simulink library "pgctrl"  (R2016b)
settings: Solver=VariableStepAuto  StartTime=0.0  StopTime=10.0  RelTol=1e-3
values from neighbouring files (symbols this model uses):
  pglfd_damping_multiplier = 1.0    (= 1)    [init_pglfd.m]
undefined symbols (not defined in the file or in its folder): curl, DiscIntNeverNeededParam, manifold_stiffness_delay_buffer_size, R3, SO3
libraries: pgctrl x24, pgmanif x15, pgtrafo x10, simulink x8, simulink_need_slupdate x1
(part 1 of 2)
settings Model: Creator=Maximilian  LastModifiedBy=mueh_mm
settings OptimizationCC: LifeSpan=inf
settings DebuggingCC: SFExecutionAtInitializationDiag=none

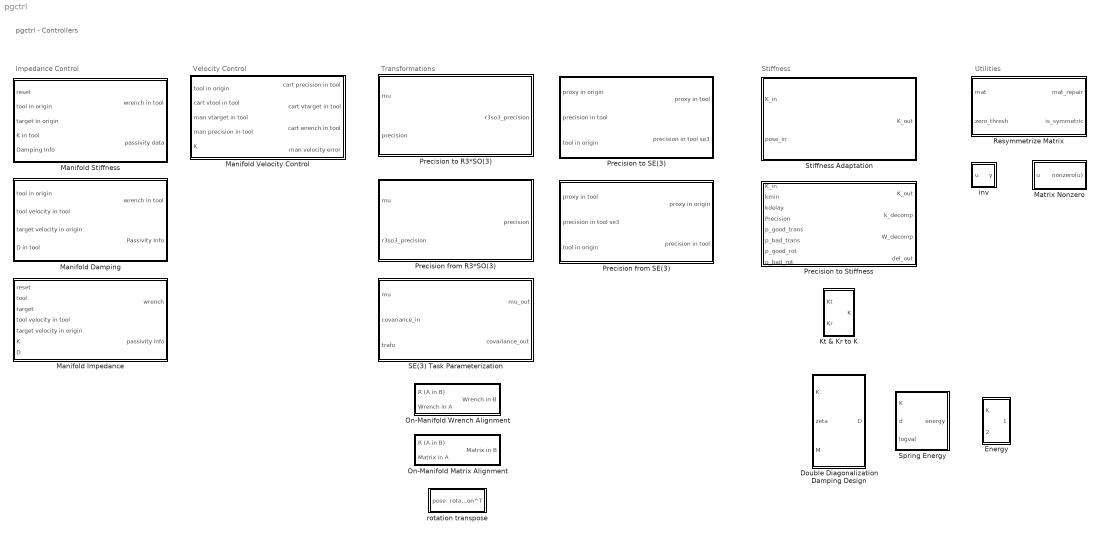
== system pgctrl ==
  note: Impedance Control
  note: pgctrl - Controllers
  note: Transformations
  note: Velocity Control
  note: Utilities
  note: Stiffness
  Double Diagonalization Damping Design : Subsystem
  Energy : Subsystem
  Kt & Kr to K : Subsystem
  Manifold Damping : Subsystem  mask(On-Manifold Damping){manifold_description_damping=R3*SO3, eps_radius=0.02}
      mask prompts: manifold_description_damping "Manifold Description"; eps_radius "Epsilon for Manifold Radius"
      mask help: This block implements the function F = D * v, generalized on the selected manifold.
      mask init:
      | % mask setup
      | mask_styles = get_param(gcb, 'MaskStyles');
      | mask_styles{1} = get_manifold_popup();
      | set_param(gcb, 'MaskStyles', mask_styles);
      | 
      | % set inside manifolds
      | set_param([gcb '/tool To Manifold'], 'manifold_description_raw', manifold_description_damping);
      | set_param([gcb '/Manifold Jacobian'], 'manifold_description_raw', manifold_description_damping);
      mask TypeOptions manifold_description_damping: SO2 | S2 | SO3 | R3*SO3 | SO2*R2*SO3 | S2*R1*SO3
      mask Display:
      | disp(['{\bf\fontsize{12}Damping}' char(10) char(10)], 'texmode','on');
      | disp([char(10) char(10) char(10) char(manifold_description_damping)]);
      | port_label('input', 1, 'tool in origin');
      | port_label('input', 2, 'vtool in tool');
      | port_label('input', 3, 'vtarget in origin');
      | port_label('input', 4, 'D in tool');
      | port_label('output', 1, 'wrench in tool');
      | port_label('output', 2, 'Passivity Info');
  Manifold Impedance : Subsystem  mask(On-Manifold Impedance){manifold_description_impedance=R3*SO3, eps_radius=0.02, passivity_method=None, initial_energy=0, initial_power=0, allow_asymmetric=off, p_active_asym=0, max_increase_passive=10}
      mask prompts: manifold_description_impedance "Manifold Description"; eps_radius "Epsilon for Manifold Radius"; passivity_method "Passivity Method"; initial_energy "Initial Energy (Joule)"; initial_power "Usage rate of initial energy (Watt)"; allow_asymmetric "Allow Asymmetric Part of Stiffness Matrix"; p_active_asym "Active power for asymmetric part"; max_increase_passive "Maximum increase of length per second"
      mask help: This block implements the function F = K * x + D * v, generalized on the selected manifold.
      mask init:
      | % mask setup
      | mask_styles = get_param(gcb, 'MaskStyles');
      | mask_styles{1} = get_manifold_popup();
      | set_param(gcb, 'MaskStyles', mask_styles);
      | 
      | % set inside manifolds
      | set_param([gcb '/Manifold Stiffness'], 'manifold_description_stiffness', manifold_description_impedance);
      | set_param([gcb '/Manifold Damping'], 'manifold_description_damping', manifold_description_impedance);
      | set_param([gcb '/Manifold Curl Stiffness/tool To Manifold'], 'manifold_description_raw', manifold_description_impedance);
      | set_param([gcb '/Manifold Curl Stiffness/Manifold Jacobian'], 'manifold_description_raw', manifold_description_impedance);
      mask TypeOptions manifold_description_impedance: SO2 | S2 | SO3 | R3*SO3 | SO2*R2*SO3 | S2*R1*SO3
      mask TypeOptions passivity_method: None | Limit delta x | Limit Kdot | Limit delta x discrete
      mask Callback passivity_method: set_param([gcb '/Manifold Stiffness'], 'passivity_method', get_param(gcb, 'passivity_method'));
      mask Display:
      | disp(['{\bf\fontsize{12}Impedance}' char(10) char(10)], 'texmode','on');
      | disp([char(10) char(10) char(10) char(manifold_description_impedance)]);
      | port_label('input', 1, 'reset');
      | port_label('input', 2, 'tool in origin');
      | port_label('input', 3, 'target in origin');
      | port_label('input', 4, 'vtool in tool');
      | port_label('input', 5, 'vtarget in origin');
      | port_label('input', 6, 'K in tool');
      | port_label('input', 7, 'D in tool');
      | port_label('output', 1, 'wrench in tool');
      | port_label('output', 2, 'passivity info');
  Manifold Stiffness : Subsystem  mask(On-Manifold Stiffness){manifold_description_stiffness=R3*SO3, eps_radius=0.02, passivity_method=None, initial_energy=0, initial_power=0, max_increase_passive=10}
      mask prompts: manifold_description_stiffness "Manifold Description"; eps_radius "Epsilon for Manifold Radius"; passivity_method "Passivity Method"; initial_energy "Initial Energy (Joule)"; initial_power "Usage rate of initial energy (Watt)"; max_increase_passive "Maximum increase of length per second"
      mask help: This block implements the function F = K * x, generalized on the selected manifold.
      mask init:
      | % mask setup
      | mask_styles = get_param(gcb, 'MaskStyles');
      | mask_styles{1} = get_manifold_popup();
      | set_param(gcb, 'MaskStyles', mask_styles);
      | 
      | % set inside manifolds
      | set_param([gcb '/target To Manifold'], 'manifold_description_raw', manifold_description_stiffness);
      | set_param([gcb '/tool To Manifold'], 'manifold_description_raw', manifold_description_stiffness);
      | set_param([gcb '/Manifold Jacobian'], 'manifold_description_raw', manifold_description_stiffness);
      | set_param([gcb '/Manifold Log'], 'manifold_description_raw', manifold_description_stiffness);
      mask TypeOptions manifold_description_stiffness: SO2 | S2 | SO3 | R3*SO3 | SO2*R2*SO3 | S2*R1*SO3
      mask TypeOptions passivity_method: None | Limit delta x | Limit Kdot | Limit delta x discrete
      mask Display:
      | disp(['{\bf\fontsize{12}Stiffness}' char(10) char(10)], 'texmode','on');
      | disp([char(10) char(10) char(10) char(manifold_description_stiffness)]);
      | port_label('input', 1, 'reset');
      | port_label('input', 2, 'tool in origin');
      | port_label('input', 3, 'target in origin');
      | port_label('input', 4, 'K in tool');
      | port_label('input', 5, 'Damping Info');
      | port_label('output', 1, 'wrench in tool');
      | port_label('output', 2, 'passivity info');
  Manifold Velocity Control : Subsystem  mask(On-Manifold Velocity Control){manifold_description_stiffness=R3*SO3, eps_radius=0.02}
      mask prompts: manifold_description_stiffness "Manifold Description"; eps_radius "Epsilon for Manifold Radius"
      mask help: This block implements the function F = K * (xref' - x'), generalized on the selected manifold. It outputs a cartesian wrench in the target frame
      mask init:
      | % mask setup
      | mask_styles = get_param(gcb, 'MaskStyles');
      | mask_styles{1} = get_manifold_popup();
      | set_param(gcb, 'MaskStyles', mask_styles);
      | 
      | % set inside manifolds
      | set_param([gcb '/tool To Manifold'], 'manifold_description_raw', manifold_description_stiffness);
      | set_param([gcb '/Manifold Jacobian'], 'manifold_description_raw', manifold_description_stiffness);
      | set_param([gcb '/Precision to SE(3)'], 'manifold_description_raw', manifold_description_stiffness);
      | set_param([gcb '/Stiffness Adaptation'], 'manifold_description_raw', manifold_description_stiffness);
      mask TypeOptions manifold_description_stiffness: SO2 | S2 | SO3 | R3*SO3 | SO2*R2*SO3 | S2*R1*SO3
      mask Display:
      | disp(['{\bf\fontsize{12}Velocity Control}' char(10) char(10)], 'texmode','on');
      | disp([char(10) char(10) char(10) char(manifold_description_stiffness)]);
      | port_label('input', 1, 'tool in origin');
      | port_label('input', 2, 'cart vtool');
      | port_label('input', 3, 'man vtarget');
      | port_label('input', 4, 'man prec');
      | port_label('input', 5, 'D');
      | port_label('output', 1, 'cart precision');
      | port_label('output', 2, 'cart vtarget');
      | port_label('output', 3, 'cart wrench');
      | port_label('output', 4, 'man velocity error');
  Matrix Nonzero : Subsystem
  On-Manifold Matrix Alignment : Subsystem
  On-Manifold Wrench Alignment : Subsystem
  Precision from R3*SO(3) : Subsystem  mask(Precision from R3*SO(3)){manifold_description_raw=R3*SO3, eps_radius=0.02}
      mask prompts: manifold_description_raw "Manifold Description"; eps_radius "Epsilon for Manifold Radius"
      mask help: This block transforms a covariance matrix from R3*SO3 to a covariance matrix on the selected manifold using the jacobian.
      mask init:
      | % mask setup
      | mask_styles = get_param(gcb, 'MaskStyles');
      | mask_styles{1} = get_manifold_popup();
      | set_param(gcb, 'MaskStyles', mask_styles);
      | 
      | % set inside manifolds
      | set_param([gcb '/To Manifold'], 'manifold_description_raw', manifold_description_raw);
      | set_param([gcb '/Manifold Jacobian'], 'manifold_description_raw', manifold_description_raw);
      mask TypeOptions manifold_description_raw: SO2 | S2 | SO3 | R3*SO3 | SO2*R2*SO3 | S2*R1*SO3
      mask Display:
      | text(0.5, 0.7, ['{\bf\fontsize{12}' char(manifold_description_raw) char(10) 'Precision}'], 'HorizontalAlignment', 'center', 'texmode', 'on');
      | disp([char(10) char(10) char(10) 'from R3*SO3']);
      | port_label('input', 1, 'mu');
      | port_label('input', 2, 'R3*SO(3) precision');
      | port_label('output', 1, 'precision');
  Precision from SE(3) : Subsystem  mask(Precision from SE(3)){manifold_description_raw=R3*SO3, eps_radius=0.02}
      mask prompts: manifold_description_raw "Manifold Description"; eps_radius "Epsilon for Manifold Radius"
      mask help: Transform a SE(3) precision matrix in tool coordinates at proxy to an on-manifold precision matrix in origin coordinates.
      mask init:
      | % mask setup
      | mask_styles = get_param(gcb, 'MaskStyles');
      | mask_styles{1} = get_manifold_popup();
      | set_param(gcb, 'MaskStyles', mask_styles);
      | 
      | % set inside manifolds
      | set_param([gcb '/Precision from R3*SO(3)'], 'manifold_description_raw', manifold_description_raw);
      mask TypeOptions manifold_description_raw: SO2 | S2 | SO3 | R3*SO3 | SO2*R2*SO3 | S2*R1*SO3
      mask Display:
      | text(0.5, 0.7, ['{\bf\fontsize{12}' char(manifold_description_raw) char(10) 'Precision}'], 'HorizontalAlignment', 'center', 'texmode', 'on');
      | disp([char(10) char(10) char(10) 'from SE(3)']);
      | port_label('input', 1, 'proxy in tool');
      | port_label('input', 2, 'precision in tool se(3)');
      | port_label('input', 3, 'tool in origin');
      | port_label('output', 1, 'proxy in origin');
      | port_label('output', 2, 'precision in tool');
  Precision to R3*SO(3) : Subsystem  mask(Precision to R3*SO(3)){manifold_description_raw=R3*SO3, eps_radius=0.02}
      mask prompts: manifold_description_raw "Manifold Description"; eps_radius "Epsilon for Manifold Radius"
      mask help: This block transforms a covariance matrix on the selected manifold to a R3*SO3 covariance matrix using the jacobian.
      mask init: same as pgctrl/Precision from R3*SO(3)
      mask TypeOptions manifold_description_raw: SO2 | S2 | SO3 | R3*SO3 | SO2*R2*SO3 | S2*R1*SO3
      mask Display:
      | text(0.5, 0.7, ['{\bf\fontsize{12}R3*SO(3)' char(10) 'Precision}'], 'HorizontalAlignment', 'center', 'texmode', 'on');
      | disp([char(10) char(10) char(10) 'from ' char(manifold_description_raw)]);
      | port_label('input', 1, 'mu');
      | port_label('input', 2, 'precision');
      | port_label('output', 1, 'R3*SO(3) precision');
  Precision to SE(3) : Subsystem  mask(Precision to SE(3)){manifold_description_raw=R3*SO3, eps_radius=0.02}
      mask prompts: manifold_description_raw "Manifold Description"; eps_radius "Epsilon for Manifold Radius"
      mask help: Transform an on-manifold precision matrix in origin coordinates at proxy to a SE(3) precision matrix in tool coordinates.
      mask init:
      | % mask setup
      | mask_styles = get_param(gcb, 'MaskStyles');
      | mask_styles{1} = get_manifold_popup();
      | set_param(gcb, 'MaskStyles', mask_styles);
      | 
      | % set inside manifolds
      | set_param([gcb '/Precision to R3*SO(3)'], 'manifold_description_raw', manifold_description_raw);
      mask TypeOptions manifold_description_raw: SO2 | S2 | SO3 | R3*SO3 | SO2*R2*SO3 | S2*R1*SO3
      mask Display:
      | text(0.5, 0.7, ['{\bf\fontsize{12}SE(3)' char(10) 'Precision}'], 'HorizontalAlignment', 'center', 'texmode', 'on');
      | disp([char(10) char(10) char(10) 'from ' char(manifold_description_raw)]);
      | port_label('input', 1, 'proxy in origin');
      | port_label('input', 2, 'precision in tool');
      | port_label('input', 3, 'tool in origin');
      | port_label('output', 1, 'proxy in tool');
      | port_label('output', 2, 'precision in tool se(3)');
  Precision to Stiffness : Subsystem  mask(Precision to Stiffness){}
      mask help: This block decomposes a precision matrix to create a stiffness matrix respecting limits.
      mask Display:
      | disp(['{\bf\fontsize{12}Precision to Stiffness}' char(10) char(10)], 'texmode','on');
      | port_label('input', 1, 'K_{diag}', 'texmode', 'on');
      | port_label('input', 2, 'k_{min}', 'texmode', 'on');
      | port_label('input', 3, 'k_{delay}', 'texmode', 'on');
      | port_label('input', 4, 'Precision');
      | port_label('input', 5, 'P_{good, trans}', 'texmode', 'on');
      | port_label('input', 6, 'P_{bad, trans}', 'texmode', 'on');
      | port_label('input', 7, 'P_{good, rot}', 'texmode', 'on');
      | port_label('input', 8, 'P_{bad, rot}', 'texmode', 'on');
      | port_label('output', 1, 'K_{adapted}', 'texmode', 'on');
      | port_label('output', 2, 'k_{decomp}', 'texmode', 'on');
      | port_label('output', 3, 'W_{decomp}', 'texmode', 'on');
      | port_label('output', 4, 'is_delay');
  Resymmetrize Matrix : MATLAB Function  TreatAsAtomicUnit=on
  SE(3) Task Parameterization : Subsystem  mask(SE(3) Task Parameterization){}
      mask help: This block transports a mean and covariance on R3*SO3 extracted in one coordinate system to another one using the SE(3) transformation trafo.
      mask Display:
      | disp(['{\bf\fontsize{12}SE(3) Task}' char(10) char(10)], 'texmode','on');
      | disp([char(10) char(10) '{\bf\fontsize{12}Parameterization}'], 'texmode','on');
      | port_label('input', 1, 'mu');
      | port_label('input', 2, 'covariance');
      | port_label('input', 3, 'trafo');
      | port_label('output', 1, 'mu');
      | port_label('output', 2, 'covariance');
  Spring Energy : Subsystem
  Stiffness Adaptation : Subsystem  mask(On-Manifold Stiffness Adaptation){manifold_description_raw=R3*SO3, manifold_description=0, manifold_id=0}
      mask prompts: manifold_description_raw "Manifold Description"
      mask help:
      | This block adapts a stiffness matrix on cylindrical or spherical manifolds to ensure stiffness doesn't get too low / too high for the rotational DoF's. Stiffness equivalent to the euclidean case with r=1 is achieved.
      |
      | Note that only diagonal stiffness matrices are supported.
      mask init:
      | % mask setup
      | mask_styles = get_param(gcb, 'MaskStyles');
      | mask_styles{1} = get_manifold_popup();
      | set_param(gcb, 'MaskStyles', mask_styles);
      | 
      | % set description
      | manifold_description = uint8(manifold_description_raw);
      | 
      | % set manifold id
      | manifold_id = 0;
      | if contains(char(manifold_description), 'SO2*R2')
      |     manifold_id = 1;
      | elseif contains(char(manifold_description), 'S2*R1')
      |     manifold_id = 2;
      | end
      mask TypeOptions manifold_description_raw: SO2 | S2 | SO3 | R3*SO3 | SO2*R2*SO3 | S2*R1*SO3
      mask Display:
      | disp(['{\bf\fontsize{12}Stiffness Adaptation}' char(10) char(10)], 'texmode','on');
      | disp([char(10) char(10) char(10) char(manifold_description)]);
      | port_label('input', 1, 'K');
      | port_label('input', 2, 'pose on manifold');
      | port_label('output', 1, 'K_{adapted}', 'texmode', 'on');
  inv : MATLAB Function  TreatAsAtomicUnit=on
  rotation transpose : Subsystem

== system pgctrl/Double Diagonalization Damping Design ==
  note: ToDo: check if M is PD
  K : Inport
  zeta : Inport  Port=2
  M : Inport  Port=3
  Constant : Constant  Value=zeros(6,6)
  Damping Design using Double Diagonalization : Subsystem
  Logical Operator : Logic  AllPortsSameDT=off  OutDataTypeStr=boolean
  Switch : Switch  Criteria=u2 > Threshold
  check finite : Subsystem
  check symmetric : Subsystem
  symmetrize : Subsystem
  D : Outport
  wires:
  check finite/1(finite) -> Logical Operator/1
  Switch/1 -> D/1
  Constant/1 -> Switch/3
  Logical Operator/1 -> Switch/2
  Damping Design using Double Diagonalization/1(D) -> Switch/1, check finite/1(matrix)
  K/1 -> symmetrize/1(K)
  check symmetric/1(is sym) -> Logical Operator/2
  M/1 -> Damping Design using Double Diagonalization/3(M), check symmetric/1(M)
  zeta/1 -> Damping Design using Double Diagonalization/2(zeta)
  symmetrize/1(Ksym) -> Damping Design using Double Diagonalization/1(K)

== system pgctrl/Energy ==
  K : Inport
  logval : Inport  Port=2
  Constant2 : Constant  Value=0.5
  Math Function2 : Math  Operator=transpose  SaturateOnIntegerOverflow=on
  Product3 : Product  Inputs=4  Multiplication=Matrix(*)
  energy : Outport
  wires:
  Math Function2/1 -> Product3/2
  Product3/1 -> energy/1
  logval/1 -> Math Function2/1, Product3/4
  K/1 -> Product3/3
  Constant2/1 -> Product3/1

== system pgctrl/Kt & Kr to K ==
  Kt : Inport
  Kr : Inport  Port=2
  Empty Stiffness : Constant  Value=zeros(6,6)
  Kr Assignment : Assignment  NumberOfDimensions=2  DiagnosticForDimensions=Warning  IndexOptions=Index vector (dialog),Index vector (dialog)  Indices=4:6,4:6  OutputSizes=1,1
  Kt Assignment : Assignment  NumberOfDimensions=2  DiagnosticForDimensions=Warning  IndexOptions=Index vector (dialog),Index vector (dialog)  Indices=1:3,1:3  OutputSizes=1,1
  K : Outport
  wires:
  Kt Assignment/1 -> Kr Assignment/1
  Kr/1 -> Kr Assignment/2
  Kr Assignment/1 -> K/1
  Kt/1 -> Kt Assignment/2
  Empty Stiffness/1 -> Kt Assignment/1

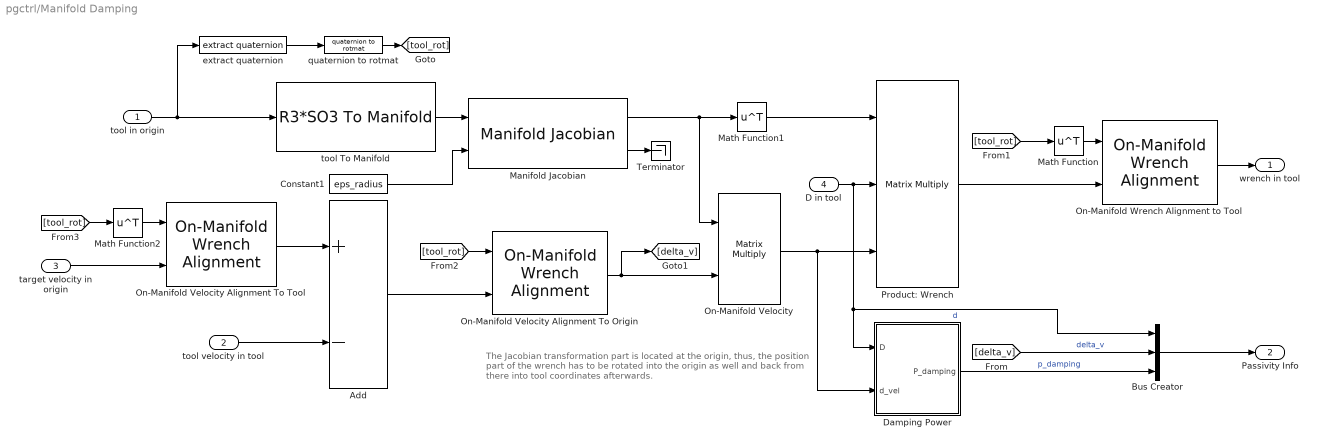
== system pgctrl/Manifold Damping ==
  note: The Jacobian transformation part is located at the origin, thus,
      | the position part of the wrench has to be rotated into the origin as well
      | and back from there into tool coordinates afterwards.
  tool in origin : Inport
  tool velocity in tool : Inport  Port=2
  target velocity in origin : Inport  Port=3
  D in tool : Inport  Port=4
  Add : Sum  Inputs=+-
  Bus Creator : BusCreator  Inputs=3
  Constant1 : Constant  Value=eps_radius
  Damping Power : Subsystem
  Manifold Jacobian : pgmanif/Manifold Jacobian  manifold_description_raw=R3*SO3  manifold_description=0  dim_manifold=0  dim_tangent=0  manifold_id=0
  Math Function : Math  Operator=transpose  SaturateOnIntegerOverflow=on
  Math Function1 : Math  Operator=transpose  SaturateOnIntegerOverflow=on
  Math Function2 : Math  Operator=transpose  SaturateOnIntegerOverflow=on
  On-Manifold Velocity : Product  Multiplication=Matrix(*)
  On-Manifold Velocity Alignment To Origin : pgctrl/On-Manifold Wrench Alignment
  On-Manifold Velocity Alignment To Tool : pgctrl/On-Manifold Wrench Alignment
  On-Manifold Wrench Alignment to Tool : pgctrl/On-Manifold Wrench Alignment
  Product: Wrench : Product  Inputs=3  Multiplication=Matrix(*)
  Terminator : Terminator
  extract quaternion : pgtrafo/extract quaternion
  quaternion to rotmat : pgtrafo/quaternion to rotmat
  tool To Manifold : pgmanif/R3*SO3 To Manifold  manifold_description_raw=R3*SO3  manifold_description=0  dim_manifold=0  dim_tangent=0
  wrench in tool : Outport
  Passivity Info : Outport  Port=2  OutDataTypeStr=Bus: bus_manifold_passivity_damping
  wires:
  tool To Manifold/1 -> Manifold Jacobian/1
  On-Manifold Wrench Alignment to Tool/1 -> wrench in tool/1
  D in tool/1 -> Bus Creator/1, Damping Power/1(D), Product: Wrench/2  "d"
  Manifold Jacobian/1 -> On-Manifold Velocity/1, Math Function1/1
  tool in origin/1 -> extract quaternion/1, tool To Manifold/1
  On-Manifold Velocity Alignment To Tool/1 -> Add/1
  [tool_rot] -> Math Function2/1
  tool velocity in tool/1 -> Add/2
  target velocity in origin/1 -> On-Manifold Velocity Alignment To Tool/2
  Product: Wrench/1 -> On-Manifold Wrench Alignment to Tool/2
  Math Function/1 -> On-Manifold Wrench Alignment to Tool/1
  [tool_rot] -> Math Function/1
  On-Manifold Velocity Alignment To Origin/1 -> [delta_v], On-Manifold Velocity/2
  [tool_rot] -> On-Manifold Velocity Alignment To Origin/1
  Add/1 -> On-Manifold Velocity Alignment To Origin/2
  quaternion to rotmat/1 -> [tool_rot]
  extract quaternion/1 -> quaternion to rotmat/1
  On-Manifold Velocity/1 -> Damping Power/2(d_vel), Product: Wrench/3
  Math Function1/1 -> Product: Wrench/1
  Constant1/1 -> Manifold Jacobian/2
  Manifold Jacobian/2 -> Terminator/1
  Damping Power/1(P_damping) -> Bus Creator/3  "p_damping"
  Bus Creator/1 -> Passivity Info/1
  [delta_v] -> Bus Creator/2  "delta_v"
  Math Function2/1 -> On-Manifold Velocity Alignment To Tool/1

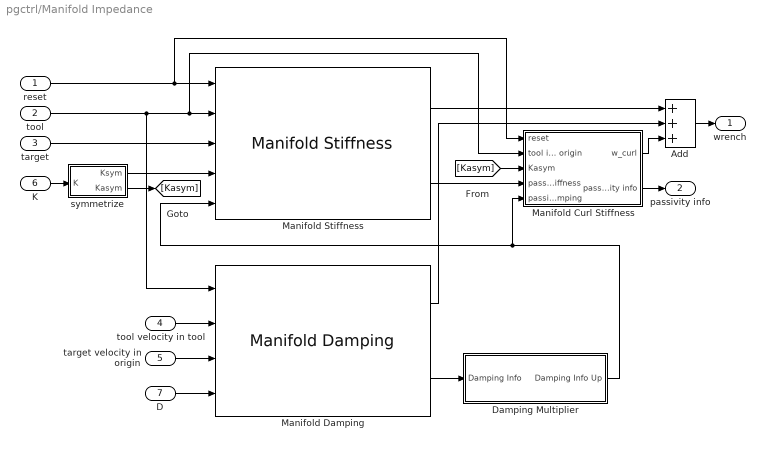
== system pgctrl/Manifold Impedance ==
  reset : Inport
  tool : Inport  Port=2
  target : Inport  Port=3
  tool velocity in tool : Inport  Port=4
  target velocity in origin : Inport  Port=5
  K : Inport  Port=6
  D : Inport  Port=7
  Add : Sum  Inputs=+++
  Damping Multiplier : Subsystem
  Manifold Curl Stiffness : Subsystem
  Manifold Damping : pgctrl/Manifold Damping  manifold_description_damping=R3*SO3  eps_radius=eps_radius
  Manifold Stiffness : pgctrl/Manifold Stiffness  manifold_description_stiffness=R3*SO3  eps_radius=eps_radius  passivity_method=None  initial_energy=initial_energy  initial_power=initial_power  max_increase_passive=max_increase_passive
  symmetrize : Subsystem
  wrench : Outport
  passivity info : Outport  Port=2
  wires:
  Manifold Stiffness/1 -> Add/1
  Manifold Damping/1 -> Add/2
  Add/1 -> wrench/1
  tool/1 -> Manifold Curl Stiffness/2(tool in origin), Manifold Stiffness/2, Manifold Damping/1
  tool velocity in tool/1 -> Manifold Damping/2
  target velocity in origin/1 -> Manifold Damping/3
  D/1 -> Manifold Damping/4
  K/1 -> symmetrize/1(K)
  target/1 -> Manifold Stiffness/3
  reset/1 -> Manifold Curl Stiffness/1(reset), Manifold Stiffness/1
  Manifold Stiffness/2 -> Manifold Curl Stiffness/4(passivity_stiffness)
  Manifold Damping/2 -> Damping Multiplier/1(Damping Info)
  Damping Multiplier/1(Damping Info Up) -> Manifold Stiffness/5, Manifold Curl Stiffness/5(passivity_damping)
  symmetrize/1(Ksym) -> Manifold Stiffness/4
  symmetrize/2(Kasym) -> [Kasym]
  Manifold Curl Stiffness/1(w_curl) -> Add/3
  [Kasym] -> Manifold Curl Stiffness/3(Kasym)
  Manifold Curl Stiffness/2(passivity info) -> passivity info/1

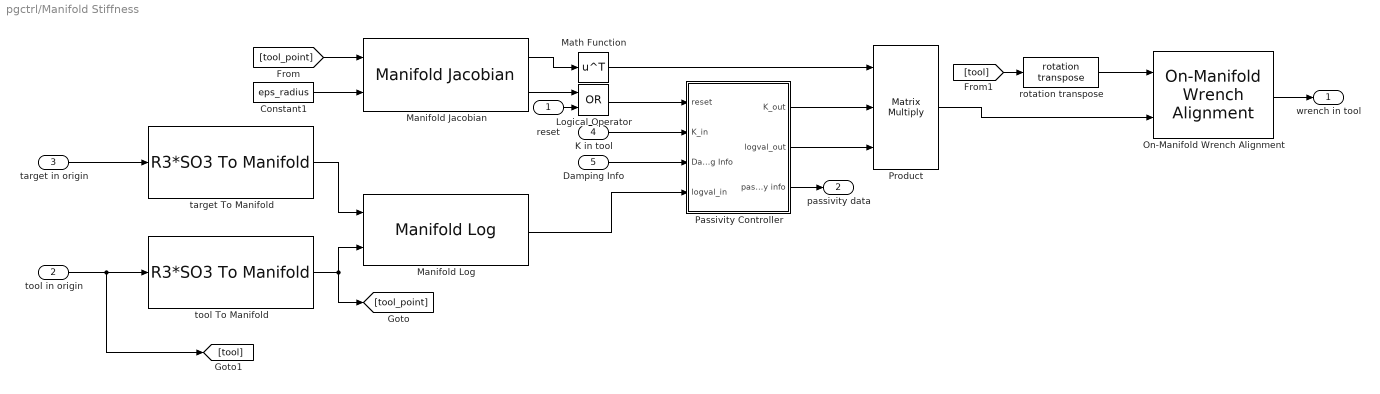
== system pgctrl/Manifold Stiffness ==
  reset : Inport
  tool in origin : Inport  Port=2
  target in origin : Inport  Port=3
  K in tool : Inport  Port=4
  Damping Info : Inport  Port=5  OutDataTypeStr=Bus: bus_manifold_passivity_damping
  Constant1 : Constant  Value=eps_radius
  Logical Operator : Logic  Operator=OR  AllPortsSameDT=off  OutDataTypeStr=boolean
  Manifold Jacobian : pgmanif/Manifold Jacobian  manifold_description_raw=R3*SO3  manifold_description=0  dim_manifold=0  dim_tangent=0  manifold_id=0
  Manifold Log : pgmanif/Manifold Log  manifold_description_raw=R3*SO3  manifold_description=0  dim_manifold=0  dim_tangent=0
  Math Function : Math  Operator=transpose  SaturateOnIntegerOverflow=on
  On-Manifold Wrench Alignment : pgctrl/On-Manifold Wrench Alignment
  Passivity Controller : Subsystem
  Product : Product  Inputs=3  Multiplication=Matrix(*)
  rotation transpose : pgctrl/rotation transpose
  target To Manifold : pgmanif/R3*SO3 To Manifold  manifold_description_raw=R3*SO3  manifold_description=0  dim_manifold=0  dim_tangent=0
  tool To Manifold : pgmanif/R3*SO3 To Manifold  manifold_description_raw=R3*SO3  manifold_description=0  dim_manifold=0  dim_tangent=0
  wrench in tool : Outport
  passivity data : Outport  Port=2
  wires:
  Product/1 -> On-Manifold Wrench Alignment/2
  target To Manifold/1 -> Manifold Log/1
  tool To Manifold/1 -> [tool_point], Manifold Log/2
  [tool_point] -> Manifold Jacobian/1
  Manifold Jacobian/1 -> Math Function/1
  target in origin/1 -> target To Manifold/1
  tool in origin/1 -> tool To Manifold/1, [tool]
  On-Manifold Wrench Alignment/1 -> wrench in tool/1
  [tool] -> rotation transpose/1
  rotation transpose/1 -> On-Manifold Wrench Alignment/1
  Math Function/1 -> Product/1
  Constant1/1 -> Manifold Jacobian/2
  K in tool/1 -> Passivity Controller/2(K_in)
  Damping Info/1 -> Passivity Controller/3(Damping Info)
  Manifold Log/1 -> Passivity Controller/4(logval_in)
  Passivity Controller/1(K_out) -> Product/2
  Passivity Controller/2(logval_out) -> Product/3
  Manifold Jacobian/2 -> Logical Operator/1
  Logical Operator/1 -> Passivity Controller/1(reset)
  reset/1 -> Logical Operator/2
  Passivity Controller/3(passivity info) -> passivity data/1

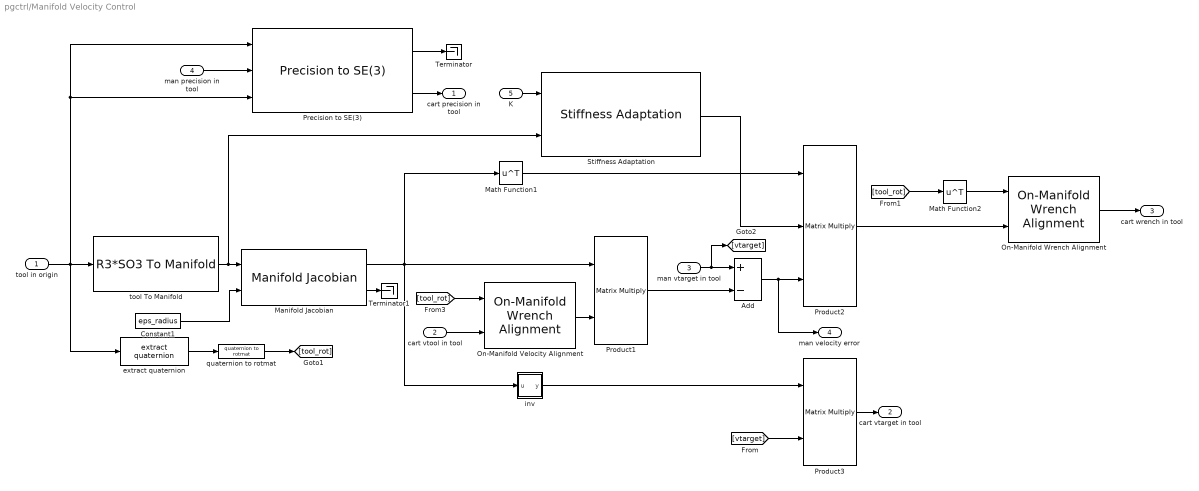
== system pgctrl/Manifold Velocity Control ==
  tool in origin : Inport
  cart vtool in tool : Inport  Port=2
  man vtarget in tool : Inport  Port=3
  man precision in tool : Inport  Port=4
  K : Inport  Port=5
  Add : Sum  Inputs=+-
  Constant1 : Constant  Value=eps_radius
  Manifold Jacobian : pgmanif/Manifold Jacobian  manifold_description_raw=R3*SO3  manifold_description=0  dim_manifold=0  dim_tangent=0  manifold_id=0
  Math Function1 : Math  Operator=transpose  SaturateOnIntegerOverflow=on
  Math Function2 : Math  Operator=transpose  SaturateOnIntegerOverflow=on
  On-Manifold Velocity Alignment : pgctrl/On-Manifold Wrench Alignment
  On-Manifold Wrench Alignment : pgctrl/On-Manifold Wrench Alignment
  Precision to SE(3) : pgctrl/Precision to SE(3)  manifold_description_raw=R3*SO3  eps_radius=eps_radius
  Product1 : Product  Multiplication=Matrix(*)
  Product2 : Product  Inputs=3  Multiplication=Matrix(*)
  Product3 : Product  Multiplication=Matrix(*)
  Stiffness Adaptation : pgctrl/Stiffness Adaptation  manifold_description_raw=R3*SO3  manifold_description=0  manifold_id=0
  Terminator : Terminator
  Terminator1 : Terminator
  extract quaternion : pgtrafo/extract quaternion
  inv : MATLAB Function  TreatAsAtomicUnit=on
  quaternion to rotmat : pgtrafo/quaternion to rotmat
  tool To Manifold : pgmanif/R3*SO3 To Manifold  manifold_description_raw=R3*SO3  manifold_description=0  dim_manifold=0  dim_tangent=0
  cart precision in tool : Outport
  cart vtarget in tool : Outport  Port=2
  cart wrench in tool : Outport  Port=3
  man velocity error : Outport  Port=4
  wires:
  [tool_rot] -> Math Function2/1
  On-Manifold Wrench Alignment/1 -> cart wrench in tool/1
  tool To Manifold/1 -> Manifold Jacobian/1, Stiffness Adaptation/2
  Manifold Jacobian/1 -> inv/1(u), Math Function1/1, Product1/1
  Product1/1 -> Add/2
  man vtarget in tool/1 -> [vtarget], Add/1
  Add/1 -> man velocity error/1, Product2/3
  Product2/1 -> On-Manifold Wrench Alignment/2
  [vtarget] -> Product3/2
  Product3/1 -> cart vtarget in tool/1
  man precision in tool/1 -> Precision to SE(3)/2
  Precision to SE(3)/2 -> cart precision in tool/1
  tool in origin/1 -> tool To Manifold/1, extract quaternion/1, Precision to SE(3)/3, Precision to SE(3)/1
  [tool_rot] -> On-Manifold Velocity Alignment/1
  cart vtool in tool/1 -> On-Manifold Velocity Alignment/2
  On-Manifold Velocity Alignment/1 -> Product1/2
  extract quaternion/1 -> quaternion to rotmat/1
  quaternion to rotmat/1 -> [tool_rot]
  K/1 -> Stiffness Adaptation/1
  Stiffness Adaptation/1 -> Product2/2
  Precision to SE(3)/1 -> Terminator/1
  Math Function1/1 -> Product2/1
  inv/1(y) -> Product3/1
  Constant1/1 -> Manifold Jacobian/2
  Math Function2/1 -> On-Manifold Wrench Alignment/1
  Manifold Jacobian/2 -> Terminator1/1

== system pgctrl/Matrix Nonzero ==
  note: Check if any of the Matrix entries is nonzero.
  u : Inport
  Matrix Nonzero : MATLAB Function  TreatAsAtomicUnit=on
  nonzero(u) : Outport
  wires:
  Matrix Nonzero/1(y) -> nonzero(u)/1
  u/1 -> Matrix Nonzero/1(u)

== system pgctrl/On-Manifold Matrix Alignment ==
  note: When computing an on-manifold matrix in a different coordinate system,
      | the positional part must be rotated accordingly: M_in_B = [R,0;0,I] M_in_A [R',0;0,I]
  R (A in B) : Inport
  Matrix in A : Inport  Port=2
  Assignment : Assignment  NumberOfDimensions=2  DiagnosticForDimensions=Warning  IndexOptions=Index vector (dialog),Index vector (dialog)  Indices=1:3,1:3  OutputSizes=1,1
  Constant : Constant  Value=eye(6)
  Math Function : Math  Operator=transpose  SaturateOnIntegerOverflow=on
  Product : Product  Inputs=3  Multiplication=Matrix(*)
  Matrix in B : Outport
  wires:
  Assignment/1 -> Math Function/1, Product/1
  R (A in B)/1 -> Assignment/2
  Constant/1 -> Assignment/1
  Product/1 -> Matrix in B/1
  Matrix in A/1 -> Product/2
  Math Function/1 -> Product/3

== system pgctrl/On-Manifold Wrench Alignment ==
  note: When computing an on-manifold wrench in a different coordinate system,
      | the forces must be rotated accordingly.
  R (A in B) : Inport
  Wrench in A : Inport  Port=2
  Product : Product  Multiplication=Matrix(*)
  Selector : Selector  InputPortWidth=6  IndexOptions=Index vector (dialog)  Indices=1:3  OutputSizes=1
  Selector1 : Selector  InputPortWidth=6  IndexOptions=Index vector (dialog)  Indices=4:6  OutputSizes=1
  Vector Concatenate : Concatenate
  Wrench in B : Outport
  wires:
  Wrench in A/1 -> Selector1/1, Selector/1
  Vector Concatenate/1 -> Wrench in B/1
  Selector/1 -> Product/2
  Selector1/1 -> Vector Concatenate/2
  Product/1 -> Vector Concatenate/1
  R (A in B)/1 -> Product/1

== system pgctrl/Precision from R3*SO(3) ==
  mu : Inport
  r3so3_precision : Inport  Port=2
  Constant1 : Constant  Value=eps_radius
  Manifold Jacobian : pgmanif/Manifold Jacobian  manifold_description_raw=R3*SO3  manifold_description=0  dim_manifold=0  dim_tangent=0  manifold_id=0
  Math Function : Math  Operator=transpose  SaturateOnIntegerOverflow=on
  Product : Product  Inputs=3  Multiplication=Matrix(*)
  To Manifold : pgmanif/R3*SO3 To Manifold  manifold_description_raw=R3*SO3  manifold_description=0  dim_manifold=0  dim_tangent=0
  inverse : MATLAB Function  TreatAsAtomicUnit=on
  precision : Outport
  wires:
  r3so3_precision/1 -> Product/2
  To Manifold/1 -> Manifold Jacobian/1
  mu/1 -> To Manifold/1
  Product/1 -> precision/1
  inverse/1(y) -> Product/1
  Manifold Jacobian/1 -> Math Function/1
  Math Function/1 -> inverse/2(u), Product/3
  Constant1/1 -> Manifold Jacobian/2
  Manifold Jacobian/2 -> inverse/1(singular)

== system pgctrl/Precision from SE(3) ==
  note: SE(3) task parametrization is needed to transform from tool to origin.
  note: Convert the precision matrix to manifold tangent coordinates from R3*SO3
      | using the manifold Jacobian.
  note: Some later calculations depend on whether the covariance is truly zero.
  proxy in tool : Inport
  precision in tool se3 : Inport  Port=2
  tool in origin : Inport  Port=3
  Constant : Constant  Value=zeros(6,6)
  Matrix Nonzero : pgctrl/Matrix Nonzero
  Precision from R3*SO(3) : pgctrl/Precision from R3*SO(3)  manifold_description_raw=R3*SO3  eps_radius=eps_radius
  SE(3) Task Parameterization : pgctrl/SE(3) Task Parameterization
  Switch : Switch  Criteria=u2 > Threshold
  proxy in origin : Outport
  precision in tool : Outport  Port=2
  wires:
  SE(3) Task Parameterization/1 -> Precision from R3*SO(3)/1, proxy in origin/1
  proxy in tool/1 -> SE(3) Task Parameterization/1
  tool in origin/1 -> SE(3) Task Parameterization/3
  Constant/1 -> Switch/3
  precision in tool se3/1 -> Matrix Nonzero/1, SE(3) Task Parameterization/2
  Matrix Nonzero/1 -> Switch/2
  Switch/1 -> precision in tool/1
  SE(3) Task Parameterization/2 -> Precision from R3*SO(3)/2
  Precision from R3*SO(3)/1 -> Switch/1

== system pgctrl/Precision to R3*SO(3) ==
  mu : Inport
  precision : Inport  Port=2
  Constant1 : Constant  Value=eps_radius
  Manifold Jacobian : pgmanif/Manifold Jacobian  manifold_description_raw=R3*SO3  manifold_description=0  dim_manifold=0  dim_tangent=0  manifold_id=0
  Math Function : Math  Operator=transpose  SaturateOnIntegerOverflow=on
  Product : Product  Inputs=3  Multiplication=Matrix(*)
  Terminator : Terminator
  To Manifold : pgmanif/R3*SO3 To Manifold  manifold_description_raw=R3*SO3  manifold_description=0  dim_manifold=0  dim_tangent=0
  r3so3_precision : Outport
  wires:
  Product/1 -> r3so3_precision/1
  mu/1 -> To Manifold/1
  To Manifold/1 -> Manifold Jacobian/1
  precision/1 -> Product/2
  Manifold Jacobian/1 -> Product/3, Math Function/1
  Math Function/1 -> Product/1
  Constant1/1 -> Manifold Jacobian/2
  Manifold Jacobian/2 -> Terminator/1

== system pgctrl/Precision to SE(3) ==
  note: Some later calculations depend on whether the covariance is truly zero.
  note: Convert the precision matrix from manifold tangent coordinates to R3*SO3
      | using the manifold Jacobian.
  note: SE(3) task parametrization is needed as the fixture arbitration happens in the toolframe.
  proxy in origin : Inport
  precision in tool : Inport  Port=2
  tool in origin : Inport  Port=3
  Constant : Constant  Value=zeros(6,6)
  Matrix Nonzero : pgctrl/Matrix Nonzero
  Precision to R3*SO(3) : pgctrl/Precision to R3*SO(3)  manifold_description_raw=R3*SO3  eps_radius=eps_radius
  SE(3) Task Parametrization : pgctrl/SE(3) Task Parameterization
  Switch : Switch  Criteria=u2 > Threshold
  invert pose : pgtrafo/invert pose
  proxy in tool : Outport
  precision in tool se3 : Outport  Port=2
  wires:
  SE(3) Task Parametrization/2 -> Switch/1
  Switch/1 -> precision in tool se3/1
  Matrix Nonzero/1 -> Switch/2
  tool in origin/1 -> Precision to R3*SO(3)/1, invert pose/1
  Precision to R3*SO(3)/1 -> SE(3) Task Parametrization/2
  Constant/1 -> Switch/3
  invert pose/1 -> SE(3) Task Parametrization/3
  proxy in origin/1 -> SE(3) Task Parametrization/1
  SE(3) Task Parametrization/1 -> proxy in tool/1
  precision in tool/1 -> Precision to R3*SO(3)/2, Matrix Nonzero/1

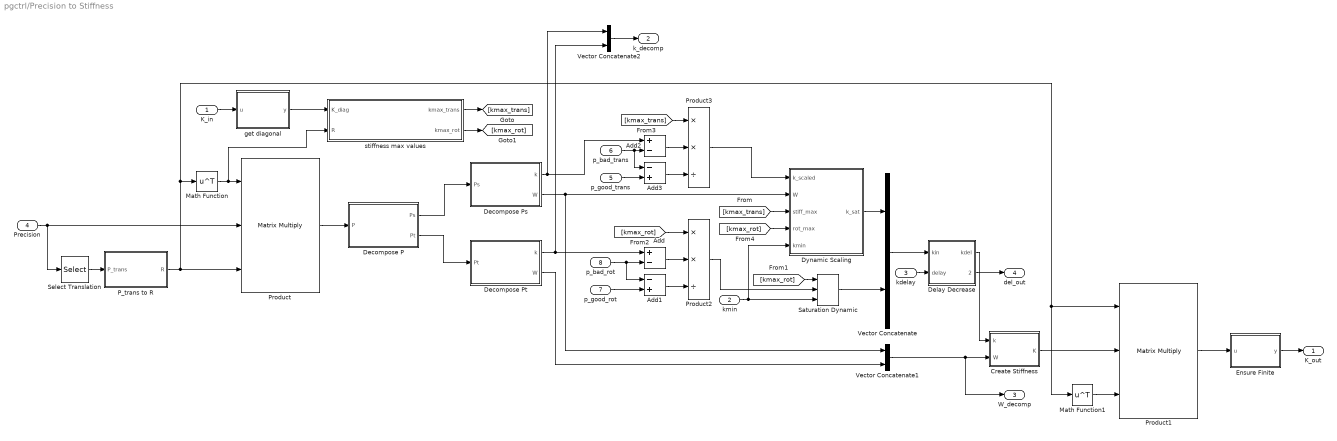
== system pgctrl/Precision to Stiffness ==
  K_in : Inport
  kmin : Inport  Port=2
  kdelay : Inport  Port=3
  Precision : Inport  Port=4
  p_good_trans : Inport  Port=5
  p_bad_trans : Inport  Port=6
  p_good_rot : Inport  Port=7
  p_bad_rot : Inport  Port=8
  Add : Sum  Inputs=+-
  Add1 : Sum  Inputs=-+
  Add2 : Sum  Inputs=+-
  Add3 : Sum  Inputs=-+
  Create Stiffness : MATLAB Function  TreatAsAtomicUnit=on
  Decompose P : MATLAB Function  TreatAsAtomicUnit=on
  Decompose Ps : MATLAB Function  TreatAsAtomicUnit=on
  Decompose Pt : MATLAB Function  TreatAsAtomicUnit=on
  Delay Decrease : Subsystem
  Dynamic Scaling : Subsystem
  Ensure Finite : MATLAB Function  TreatAsAtomicUnit=on
  Math Function : Math  Operator=transpose  SaturateOnIntegerOverflow=on
  Math Function1 : Math  Operator=transpose  SaturateOnIntegerOverflow=on
  P_trans to R : MATLAB Function  TreatAsAtomicUnit=on
  Product : Product  Inputs=3  Multiplication=Matrix(*)
  Product1 : Product  Inputs=3  Multiplication=Matrix(*)
  Product2 : Product  Inputs=**/
  Product3 : Product  Inputs=**/
  Saturation Dynamic : simulink/Discontinuities/Saturation Dynamic  OutMin=[]  OutMax=[]  OutDataTypeStr=Inherit: Same as second input  OutDataType=fixdt(1, 16)  OutScaling=2^-10  DoSatur=off
  Select Translation : Selector  NumberOfDimensions=2  InputPortWidth=3  IndexOptions=Index vector (dialog),Index vector (dialog)  Indices=1:3,1:3  OutputSizes=1,1
  Vector Concatenate : Concatenate
  Vector Concatenate1 : Concatenate  Mode=Multidimensional array  ConcatenateDimension=2
  Vector Concatenate2 : Concatenate  Mode=Multidimensional array
  get diagonal : MATLAB Function  TreatAsAtomicUnit=on
  stiffness max values : MATLAB Function  TreatAsAtomicUnit=on
  K_out : Outport
  k_decomp : Outport  Port=2
  W_decomp : Outport  Port=3
  del_out : Outport  Port=4
  wires:
  Precision/1 -> Product/2, Select Translation/1
  Decompose P/1(Ps) -> Decompose Ps/1(Ps)
  Decompose P/2(Pt) -> Decompose Pt/1(Pt)
  Select Translation/1 -> P_trans to R/1(P_trans)
  P_trans to R/1(R) -> Math Function/1, Product1/1, Math Function1/1, Product/3
  Product/1 -> Decompose P/1(P)
  Decompose Pt/1(k) -> Vector Concatenate2/2, Add/1
  Decompose Pt/2(W) -> Vector Concatenate1/2
  Decompose Ps/2(W) -> Vector Concatenate1/1, Dynamic Scaling/2(W)
  Vector Concatenate1/1 -> W_decomp/1, Create Stiffness/2(W)
  Create Stiffness/1(K) -> Product1/2
  Product1/1 -> Ensure Finite/1(u)
  Product2/1 -> Saturation Dynamic/2
  Math Function/1 -> stiffness max values/2(R), Product/1
  Math Function1/1 -> Product1/3
  Ensure Finite/1(y) -> K_out/1
  Saturation Dynamic/1 -> Vector Concatenate/2
  [kmax_rot] -> Saturation Dynamic/1
  kmin/1 -> Dynamic Scaling/5(kmin), Saturation Dynamic/3
  Dynamic Scaling/1(k_sat) -> Vector Concatenate/1
  Product3/1 -> Dynamic Scaling/1(k_scaled)
  [kmax_trans] -> Dynamic Scaling/3(stiff_max)
  K_in/1 -> get diagonal/1(u)
  get diagonal/1(y) -> stiffness max values/1(K_diag)
  stiffness max values/1(kmax_trans) -> [kmax_trans]
  stiffness max values/2(kmax_rot) -> [kmax_rot]
  p_bad_rot/1 -> Add1/1, Add/2
  Add/1 -> Product2/2
  p_good_rot/1 -> Add1/2
  Add1/1 -> Product2/3
  [kmax_rot] -> Product2/1
  Decompose Ps/1(k) -> Add2/1, Vector Concatenate2/1
  p_bad_trans/1 -> Add3/1, Add2/2
  Add2/1 -> Product3/2
  p_good_trans/1 -> Add3/2
  Add3/1 -> Product3/3
  [kmax_trans] -> Product3/1
  [kmax_rot] -> Dynamic Scaling/4(rot_max)
  Vector Concatenate2/1 -> k_decomp/1
  kdelay/1 -> Delay Decrease/2(delay)
  Vector Concatenate/1 -> Delay Decrease/1(kin)
  Delay Decrease/1(kdel) -> Create Stiffness/1(k)
  Delay Decrease/2(del_out) -> del_out/1

== system pgctrl/SE(3) Task Parameterization ==
  mu : Inport
  covariance_in : Inport  Port=2
  trafo : Inport  Port=3
  R3*SO3 Task Parameterization : pgmanif/R3*SO3 Task Parameterization  manifold_description=SO2  dim_tangent=0  dim_manifold=0
  SE(3) Rotation : Subsystem
  mu_out : Outport
  covariance_out : Outport  Port=2
  wires:
  mu/1 -> R3*SO3 Task Parameterization/1
  covariance_in/1 -> R3*SO3 Task Parameterization/2
  R3*SO3 Task Parameterization/1 -> mu_out/1
  R3*SO3 Task Parameterization/2 -> covariance_out/1
  trafo/1 -> R3*SO3 Task Parameterization/4, SE(3) Rotation/1(trafo)
  SE(3) Rotation/1(rot) -> R3*SO3 Task Parameterization/3

== system pgctrl/Spring Energy ==
  K : Inport
  d : Inport  Port=2
  logval : Inport  Port=3
  Constant : Constant  Value=0.5
  Math Function : Math  Operator=transpose  SaturateOnIntegerOverflow=on
  Product : Product  Inputs=6  Multiplication=Matrix(*)
  energy : Outport
  wires:
  Constant/1 -> Product/1
  d/1 -> Product/3, Product/2
  Math Function/1 -> Product/4
  logval/1 -> Product/6, Math Function/1
  K/1 -> Product/5
  Product/1 -> energy/1

== system pgctrl/Stiffness Adaptation ==
  K_in : Inport
  pose_in : Inport  Port=2
  Stiffness Adaptation : MATLAB Function  TreatAsAtomicUnit=on
  K_out : Outport
  wires:
  K_in/1 -> Stiffness Adaptation/1(Kin)
  Stiffness Adaptation/1(Kadap) -> K_out/1
  pose_in/1 -> Stiffness Adaptation/2(pose_in)

== system pgctrl/rotation transpose ==
  pose : Inport
  Math Function : Math  Operator=transpose  SaturateOnIntegerOverflow=on
  extract quaternion : pgtrafo/extract quaternion
  quaternion to rotmat : pgtrafo/quaternion to rotmat
  rotation^T : Outport
  wires:
  quaternion to rotmat/1 -> Math Function/1
  Math Function/1 -> rotation^T/1
  pose/1 -> extract quaternion/1
  extract quaternion/1 -> quaternion to rotmat/1

== system pgctrl/Double Diagonalization Damping Design/Damping Design using Double Diagonalization ==
  note: A. Albu-Schaffer, C. Ott, U. Frese and G. Hirzinger,
      | "Cartesian impedance control of redundant robots: recent results with the DLR-light-weight-arms,"
      | 2003 IEEE International Conference on Robotics and Automation (Cat. No.03CH37422) ,
      | Taipei, Taiwan, 2003, pp. 3704-3709 vol.3, doi: 10.1109/ROBOT.2003.1242165.
  K : Inport
  zeta : Inport  Port=2
  M : Inport  Port=3
  Damping Design : MATLAB Function  TreatAsAtomicUnit=on
  D : Outport
  wires:
  K/1 -> Damping Design/1(K)
  M/1 -> Damping Design/2(M)
  zeta/1 -> Damping Design/3(zeta)
  Damping Design/1(D) -> D/1

== system pgctrl/Double Diagonalization Damping Design/check finite ==
  matrix : Inport
  Logical Operator1 : Logic  Inputs=1  AllPortsSameDT=off  OutDataTypeStr=boolean
  Relational Operator1 : RelationalOperator  Operator=isFinite  OutDataTypeStr=boolean  RndMeth=Nearest
  Reshape : Reshape
  finite : Outport
  wires:
  Reshape/1 -> Logical Operator1/1
  Logical Operator1/1 -> finite/1
  Relational Operator1/1 -> Reshape/1
  matrix/1 -> Relational Operator1/1

== system pgctrl/Double Diagonalization Damping Design/check symmetric ==
  M : Inport
  Abs : Abs
  Add4 : Sum  Inputs=+-
  Compare To Constant : simulink/Logic and Bit Operations/Compare To Constant  relop=<=  const=1e-8  OutDataTypeStr=boolean
  Math Function1 : Math  Operator=transpose  SaturateOnIntegerOverflow=on
  Sum of Elements : Sum  Inputs=+
  is sym : Outport
  wires:
  Abs/1 -> Sum of Elements/1
  Sum of Elements/1 -> Compare To Constant/1
  M/1 -> Add4/1, Math Function1/1
  Math Function1/1 -> Add4/2
  Add4/1 -> Abs/1
  Compare To Constant/1 -> is sym/1

== system pgctrl/Double Diagonalization Damping Design/symmetrize ==
  K : Inport
  Add : Sum
  Gain : Gain  Gain=0.5
  Math Function : Math  Operator=transpose  SaturateOnIntegerOverflow=on
  Ksym : Outport
  wires:
  Add/1 -> Gain/1
  Gain/1 -> Ksym/1
  Math Function/1 -> Add/2
  K/1 -> Math Function/1, Add/1

== system pgctrl/Manifold Damping/Damping Power ==
  D : Inport
  d_vel : Inport  Port=2
  Math Function : Math  Operator=transpose  SaturateOnIntegerOverflow=on
  Product : Product  Inputs=3  Multiplication=Matrix(*)
  P_damping : Outport
  wires:
  d_vel/1 -> Product/3, Math Function/1
  Math Function/1 -> Product/1
  D/1 -> Product/2
  Product/1 -> P_damping/1

== system pgctrl/Manifold Impedance/Damping Multiplier ==
  Damping Info : Inport
  Bus Assignment : BusAssignment  AssignedSignals=p_damping
  Bus Selector : BusSelector  OutputSignals=p_damping
  Constant : Constant  Value=pglfd_damping_multiplier
  Product : Product
  Damping Info Up : Outport
  wires:
  Damping Info/1 -> Bus Assignment/1, Bus Selector/1
  Product/1 -> Bus Assignment/2
  Bus Assignment/1 -> Damping Info Up/1
  Bus Selector/1 -> Product/1  "<p_damping>"
  Constant/1 -> Product/2

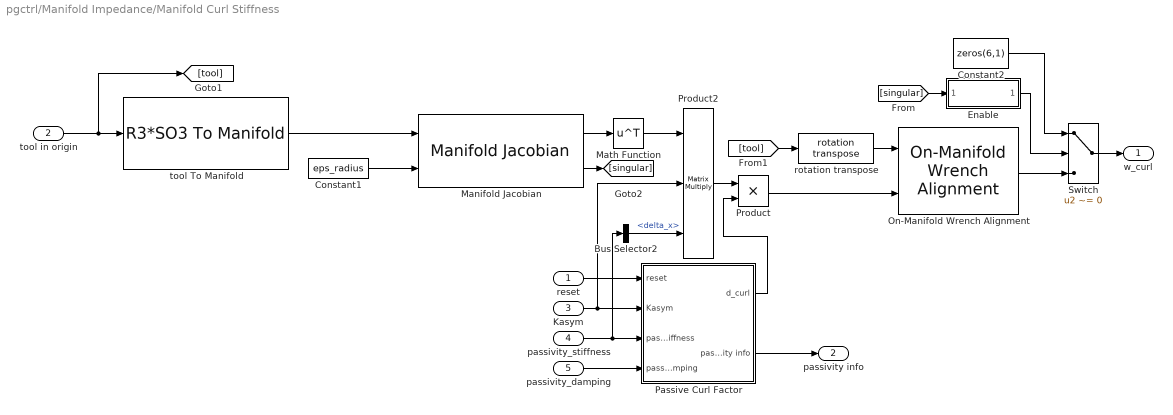
== system pgctrl/Manifold Impedance/Manifold Curl Stiffness ==
  reset : Inport
  tool in origin : Inport  Port=2
  Kasym : Inport  Port=3
  passivity_stiffness : Inport  Port=4
  passivity_damping : Inport  Port=5
  Bus Selector2 : BusSelector  OutputSignals=computed.delta_x
  Constant1 : Constant  Value=eps_radius
  Constant2 : Constant  Value=zeros(6,1)
  Enable : Subsystem
  Manifold Jacobian : pgmanif/Manifold Jacobian  manifold_description_raw=R3*SO3  manifold_description=0  dim_manifold=0  dim_tangent=0  manifold_id=0
  Math Function : Math  Operator=transpose  SaturateOnIntegerOverflow=on
  On-Manifold Wrench Alignment : pgctrl/On-Manifold Wrench Alignment
  Passive Curl Factor : Subsystem
  Product : Product
  Product2 : Product  Inputs=3  Multiplication=Matrix(*)
  Switch : Switch  Criteria=u2 ~= 0
  rotation transpose : pgctrl/rotation transpose
  tool To Manifold : pgmanif/R3*SO3 To Manifold  manifold_description_raw=R3*SO3  manifold_description=R3*SO3  dim_manifold=0  dim_tangent=0
  w_curl : Outport
  passivity info : Outport  Port=2
  wires:
  passivity_damping/1 -> Passive Curl Factor/4(passivity_damping)
  passivity_stiffness/1 -> Bus Selector2/1, Passive Curl Factor/3(passivity_stiffness)
  Kasym/1 -> Product2/2, Passive Curl Factor/2(Kasym)
  Bus Selector2/1 -> Product2/3  "<delta_x>"
  Constant1/1 -> Manifold Jacobian/2
  rotation transpose/1 -> On-Manifold Wrench Alignment/1
  [tool] -> rotation transpose/1
  tool in origin/1 -> [tool], tool To Manifold/1
  Manifold Jacobian/1 -> Math Function/1
  tool To Manifold/1 -> Manifold Jacobian/1
  Product/1 -> On-Manifold Wrench Alignment/2
  Math Function/1 -> Product2/1
  Product2/1 -> Product/1
  Passive Curl Factor/1(d_curl) -> Product/2
  Constant2/1 -> Switch/1
  Manifold Jacobian/2 -> [singular]
  [singular] -> Enable/1(singular)
  Enable/1(enable) -> Switch/2
  On-Manifold Wrench Alignment/1 -> Switch/3
  Switch/1 -> w_curl/1
  Passive Curl Factor/2(passivity info) -> passivity info/1
  reset/1 -> Passive Curl Factor/1(reset)

== system pgctrl/Manifold Impedance/symmetrize ==
  K : Inport
  Add : Sum
  Add1 : Sum  Inputs=+-
  Gain : Gain  Gain=0.5
  Gain1 : Gain  Gain=0.5
  Math Function : Math  Operator=transpose  SaturateOnIntegerOverflow=on
  Ksym : Outport
  Kasym : Outport  Port=2
  wires:
  Add/1 -> Gain/1
  Gain/1 -> Ksym/1
  Math Function/1 -> Add1/2, Add/2
  K/1 -> Math Function/1, Add1/1, Add/1
  Gain1/1 -> Kasym/1
  Add1/1 -> Gain1/1

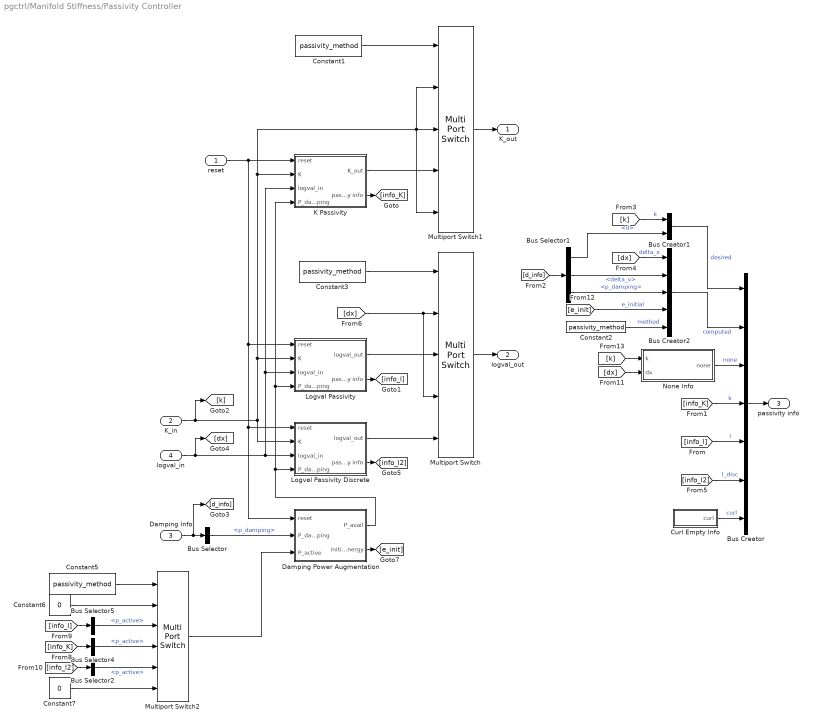
== system pgctrl/Manifold Stiffness/Passivity Controller ==
  reset : Inport
  K_in : Inport  Port=2
  Damping Info : Inport  Port=3
  logval_in : Inport  Port=4
  Bus Creator : BusCreator  Inputs=7  OutDataTypeStr=Bus: bus_manifold_passivity_info  NonVirtualBus=on
  Bus Creator1 : BusCreator  Inputs=2  OutDataTypeStr=Bus: bus_manifold_passivity_desired
  Bus Creator2 : BusCreator  Inputs=5  OutDataTypeStr=Bus: bus_manifold_passivity_computed
  Bus Selector : BusSelector  OutputSignals=p_damping
  Bus Selector1 : BusSelector  OutputSignals=d,delta_v,p_damping
  Bus Selector2 : BusSelector  OutputSignals=p_active
  Bus Selector4 : BusSelector  OutputSignals=p_active
  Bus Selector5 : BusSelector  OutputSignals=p_active
  Constant1 : Constant  Value=passivity_method
  Constant2 : Constant  Value=passivity_method  OutDataTypeStr=uint8
  Constant3 : Constant  Value=passivity_method
  Constant5 : Constant  Value=passivity_method
  Constant6 : Constant  Value=0
  Constant7 : Constant  Value=0
  Curl Empty Info : Subsystem
  Damping Power Augmentation : Subsystem
  K Passivity : Subsystem
  Logval Passivity : Subsystem
  Logval Passivity Discrete : Subsystem
  Multiport Switch : MultiPortSwitch  Inputs=4  DiagnosticForDefault=Warning
  Multiport Switch1 : MultiPortSwitch  Inputs=4  DiagnosticForDefault=Warning
  Multiport Switch2 : MultiPortSwitch  Inputs=5  DiagnosticForDefault=Warning
  None Info : Subsystem
  K_out : Outport
  logval_out : Outport  Port=2
  passivity info : Outport  Port=3  OutDataTypeStr=Bus: bus_manifold_passivity_info
  wires:
  logval_in/1 -> K Passivity/3(logval_in), Logval Passivity/3(logval_in), Logval Passivity Discrete/3(logval_in), [dx]
  Damping Power Augmentation/1(P_avail) -> K Passivity/4(P_damping), Logval Passivity/4(P_damping), Logval Passivity Discrete/4(P_damping)
  K_in/1 -> [k], K Passivity/2(K), Multiport Switch1/2, Multiport Switch1/3, Multiport Switch1/5, Logval Passivity/2(K), Logval Passivity Discrete/2(K)
  Logval Passivity/1(logval_out) -> Multiport Switch/3
  K Passivity/1(K_out) -> Multiport Switch1/4
  reset/1 -> Damping Power Augmentation/1(reset), Logval Passivity Discrete/1(reset), Logval Passivity/1(reset), K Passivity/1(reset)
  K Passivity/2(passivity info) -> [info_K]
  Logval Passivity/2(passivity info) -> [info_l]
  [info_K] -> Bus Creator/4  "k"
  [info_l] -> Bus Creator/5  "l"
  Bus Creator/1 -> passivity info/1
  Multiport Switch/1 -> logval_out/1
  Damping Info/1 -> [d_info], Bus Selector/1
  [k] -> Bus Creator1/1  "k"
  [d_info] -> Bus Selector1/1
  Bus Selector1/1 -> Bus Creator1/2  "<d>"
  Bus Creator1/1 -> Bus Creator/1  "desired"
  Bus Creator2/1 -> Bus Creator/2  "computed"
  [dx] -> Bus Creator2/1  "delta_x"
  Bus Selector1/2 -> Bus Creator2/2  "<delta_v>"
  Bus Selector1/3 -> Bus Creator2/3  "<p_damping>"
  Constant2/1 -> Bus Creator2/5  "method"
  [info_l2] -> Bus Creator/6  "l_disc"
  Logval Passivity Discrete/2(passivity info) -> [info_l2]
  [dx] -> Multiport Switch/2, Multiport Switch/4
  Constant3/1 -> Multiport Switch/1
  Logval Passivity Discrete/1(logval_out) -> Multiport Switch/5
  Multiport Switch1/1 -> K_out/1
  Constant1/1 -> Multiport Switch1/1
  Bus Selector/1 -> Damping Power Augmentation/2(P_damping)  "<p_damping>"
  Constant5/1 -> Multiport Switch2/1
  Constant6/1 -> Multiport Switch2/2
  [info_l] -> Bus Selector5/1
  [info_K] -> Bus Selector4/1
  [info_l2] -> Bus Selector2/1
  Bus Selector2/1 -> Multiport Switch2/5  "<p_active>"
  Bus Selector4/1 -> Multiport Switch2/4  "<p_active>"
  Bus Selector5/1 -> Multiport Switch2/3  "<p_active>"
  Multiport Switch2/1 -> Damping Power Augmentation/3(P_active)
  Damping Power Augmentation/2(initial_energy) -> [e_init]
  [e_init] -> Bus Creator2/4  "e_initial"
  Constant7/1 -> Multiport Switch2/6
  Curl Empty Info/1(curl) -> Bus Creator/7  "curl"
  None Info/1(none) -> Bus Creator/3  "none"
  [dx] -> None Info/2(dx)
  [k] -> None Info/1(k)
